simulink model "testrun"  (R2024b)
settings: Solver=FixedStepDiscrete  StartTime=0.0  StopTime=10.0  FixedStep=0.01  RelTol=1e-3  EnableMultiTasking=on
libraries: BalRobTbx_baselib x5
settings Model: ExtModeTrigDuration=2  Creator=aboulenien  LastModifiedBy=aboulenien
settings SolverCC: AutoInsertRateTranBlk=on
settings OptimizationCC: EnhancedBackFolding=on  PassReuseOutputArgsAs=Individual arguments  ZeroExternalMemoryAtStartup=off  ZeroInternalMemoryAtStartup=off  MaxStackSize=64  OptimizeBlockOrder=speed  DifferentSizesBufferReuse=on  OptimizationCustomize=off  EfficientTunableParamExpr=on
settings DebuggingCC: ParameterTunabilityLossMsg=error
settings HardwareCC: ProdBitPerInt=16  ProdBitPerPointer=16  ProdBitPerSizeT=16  ProdBitPerPtrDiffT=16  ProdLargestAtomicFloat=None  ProdWordSize=8  ProdHWDeviceType=Atmel->AVR
settings SFSimCC: MATLABDynamicMemAlloc=off
settings RTWCC: Description=Embedded Coder  SystemTargetFile=ert.tlc  HardwareBoard=Arduino Mega 2560  TemplateMakefile=ert_default_tmf  Toolchain=Arduino AVR  BuildConfiguration=Faster Runs
settings CodeAppCC: ForceParamTrailComments=on  IgnoreCustomStorageClasses=off  OperatorAnnotations=on  SimulinkDataObjDesc=on  SFDataObjDesc=on  InsertBlockDesc=on
settings ERTTargetCC: SupportContinuousTime=on  SupportVariableSizeSignals=on  ExtModeTransport=3  ExtModeStaticAlloc=on  ExtModeAutomaticAllocSize=off  ExtModeStaticAllocSize=2048  ExtModeMexFile=ext_xcp  ExtModeIntrfLevel=Level2 - Open  InlinedParameterPlacement=Hierarchical

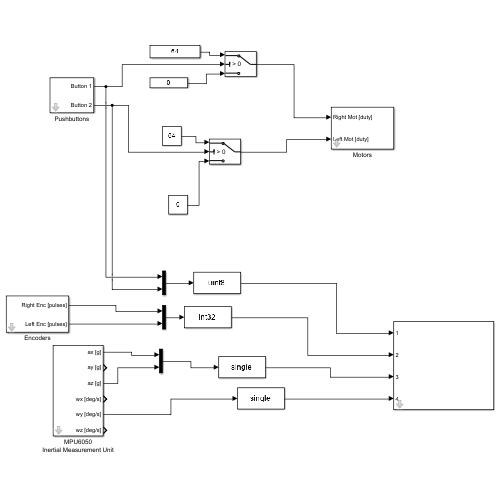
[thumbnail: Simulink's stored preview of the top-level diagram]
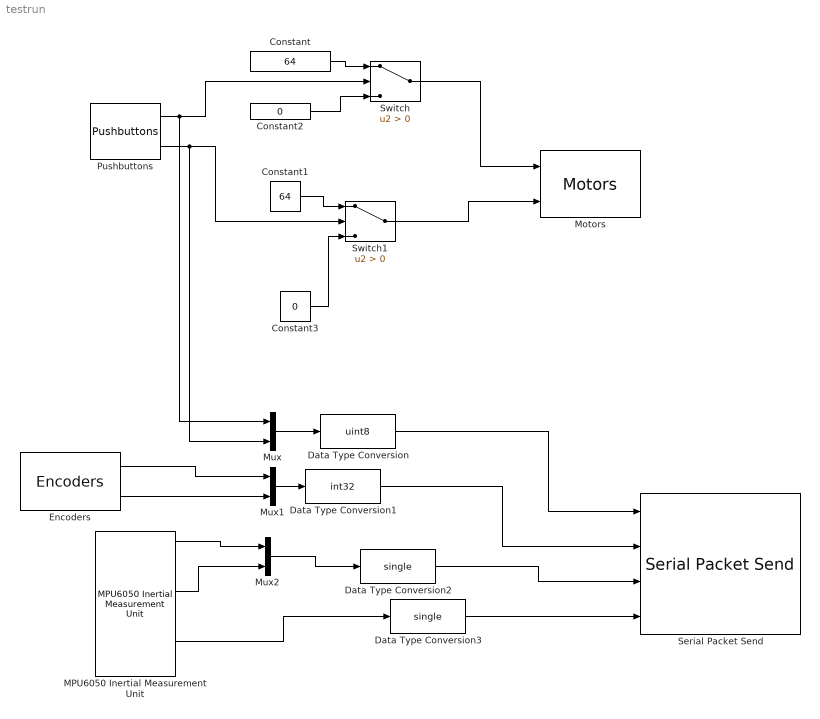
== system testrun ==
  Constant : Constant  Value=64
  Constant1 : Constant  Value=64
  Constant2 : Constant  Value=0
  Constant3 : Constant  Value=0
  Data Type Conversion : DataTypeConversion  OutDataTypeStr=uint8  SaturateOnIntegerOverflow=off  RndMeth=Floor
  Data Type Conversion1 : DataTypeConversion  OutDataTypeStr=int32  SaturateOnIntegerOverflow=off  RndMeth=Floor
  Data Type Conversion2 : DataTypeConversion  OutDataTypeStr=single  SaturateOnIntegerOverflow=off  RndMeth=Floor
  Data Type Conversion3 : DataTypeConversion  OutDataTypeStr=single  SaturateOnIntegerOverflow=off  RndMeth=Floor
  Encoders : BalRobTbx_baselib/Inputs/Encoders
      settings: SourceProductName=Balancing Robot Toolbox
  MPU6050 Inertial Measurement Unit : BalRobTbx_baselib/Inputs/MPU6050 Inertial Measurement Unit
      settings: SourceProductName=Balancing Robot Toolbox
  Motors : BalRobTbx_baselib/Outputs/Motors
      settings: SourceProductName=Balancing Robot Toolbox
  Mux : Mux  Inputs=2
  Mux1 : Mux  Inputs=2
  Mux2 : Mux  Inputs=2
  Pushbuttons : BalRobTbx_baselib/Inputs/Pushbuttons
      settings: SourceProductName=Balancing Robot Toolbox
  Serial Packet Send : BalRobTbx_baselib/Communication/Serial Packet Send  serialLinkOpt=Bluetooth  baudRateOpt=38400  waitHostTxCmd=on  txStartCmd=65  txStopCmd=66  packetSpec={'2*uint8', '2*int32', '2*single', 'single'}  cobsEncoded=on  nullTerminated=on  showEnablePort=off
      settings: SourceProductName=Balancing Robot Toolbox
  Switch : Switch  Criteria=u2 > Threshold  SaturateOnIntegerOverflow=off  InputSameDT=off
  Switch1 : Switch  Criteria=u2 > Threshold  SaturateOnIntegerOverflow=off  InputSameDT=off
  wires:
  Constant/1 -> Switch/1
  Constant2/1 -> Switch/3
  Constant1/1 -> Switch1/1
  Constant3/1 -> Switch1/3
  Pushbuttons/1 -> Mux/1, Switch/2
  Pushbuttons/2 -> Mux/2, Switch1/2
  Switch/1 -> Motors/1
  Switch1/1 -> Motors/2
  Mux/1 -> Data Type Conversion/1
  Data Type Conversion/1 -> Serial Packet Send/1
  Encoders/2 -> Mux1/2
  Encoders/1 -> Mux1/1
  Mux1/1 -> Data Type Conversion1/1
  Data Type Conversion1/1 -> Serial Packet Send/2
  MPU6050 Inertial Measurement Unit/1 -> Mux2/1
  MPU6050 Inertial Measurement Unit/3 -> Mux2/2
  Mux2/1 -> Data Type Conversion2/1
  Data Type Conversion2/1 -> Serial Packet Send/3
  MPU6050 Inertial Measurement Unit/5 -> Data Type Conversion3/1
  Data Type Conversion3/1 -> Serial Packet Send/4
